simulink model "Sistema_Control_05"  (R2026a)
settings: Solver=VariableStepAuto
settings Model: Creator=Lorenzo  LastModifiedBy=Lorenzo

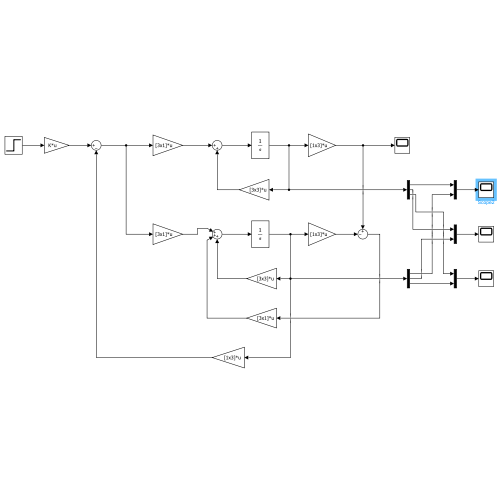
[thumbnail: Simulink's stored preview of the top-level diagram]
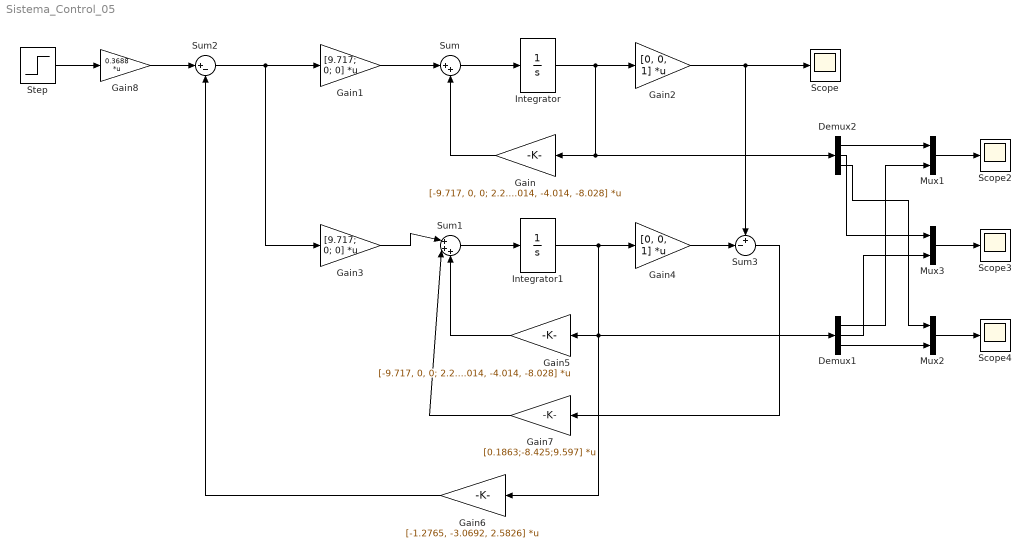
== system Sistema_Control_05 ==
  Demux1 : Demux  Outputs=3
  Demux2 : Demux  Outputs=3
  Gain : Gain  Gain=[-9.717, 0, 0; 2.209, -6.658, -2.209; 4.014, -4.014, -8.028]  Multiplication=Matrix(K*u)
  Gain1 : Gain  Gain=[9.717; 0; 0]  Multiplication=Matrix(K*u)
  Gain2 : Gain  Gain=[0, 0, 1]  Multiplication=Matrix(K*u)
  Gain3 : Gain  Gain=[9.717; 0; 0]  Multiplication=Matrix(K*u)
  Gain4 : Gain  Gain=[0, 0, 1]  Multiplication=Matrix(K*u)
  Gain5 : Gain  Gain=[-9.717, 0, 0; 2.209, -6.658, -2.209; 4.014, -4.014, -8.028]  Multiplication=Matrix(K*u)
  Gain6 : Gain  Gain=[-1.2765, -3.0692, 2.5826]  Multiplication=Matrix(K*u)
  Gain7 : Gain  Gain=[0.1863;-8.425;9.597]  Multiplication=Matrix(K*u)
  Gain8 : Gain  Gain=0.3688  Multiplication=Matrix(K*u)
  Integrator : Integrator  InitialCondition=[0;0;0]
  Integrator1 : Integrator  InitialCondition=[0.5; -0.2; 0.1]
  Mux1 : Mux  Inputs=2
  Mux2 : Mux  Inputs=2
  Mux3 : Mux  Inputs=2
  Scope{,2..4} (4 alike) : Scope
      Scope settings: ActiveDisplayYMinimum=-1  ActiveDisplayYMaximum=1
      Scope2 settings: ActiveDisplayYMinimum=-0.48021325737375165  ActiveDisplayYMaximum=2.9819512776253032  DataLoggingVariableName=ScopeData2
      Scope3 settings: ActiveDisplayYMinimum=-1  ActiveDisplayYMaximum=1  DataLoggingVariableName=ScopeData3
      Scope4 settings: ActiveDisplayYMinimum=-0.015340297796017775  ActiveDisplayYMaximum=0.12374667488104585  DataLoggingVariableName=ScopeData4
  Step : Step  SampleTime=0
  Sum : Sum  Inputs=|++
  Sum1 : Sum  Inputs=|+++
  Sum2 : Sum  Inputs=|+-
  Sum3 : Sum  Inputs=+-|
  wires:
  Gain7/1 -> Sum1/2
  Demux2/3 -> Mux2/1
  Mux3/1 -> Scope3/1
  Demux2/2 -> Mux3/1
  Demux1/2 -> Mux3/2
  Gain2/1 -> Sum3/1, Scope/1
  Integrator1/1 -> Gain6/1, Demux1/1, Gain5/1, Gain4/1
  Gain5/1 -> Sum1/3
  Sum1/1 -> Integrator1/1
  Gain1/1 -> Sum/1
  Integrator/1 -> Gain/1, Demux2/1, Gain2/1
  Demux2/1 -> Mux1/1
  Sum/1 -> Integrator/1
  Demux1/3 -> Mux2/2
  Sum3/1 -> Gain7/1
  Mux2/1 -> Scope4/1
  Gain/1 -> Sum/2
  Gain3/1 -> Sum1/1
  Demux1/1 -> Mux1/2
  Mux1/1 -> Scope2/1
  Gain4/1 -> Sum3/2
  Sum2/1 -> Gain3/1, Gain1/1
  Gain6/1 -> Sum2/2
  Gain8/1 -> Sum2/1
  Step/1 -> Gain8/1
